simulink library "Steer_Rack_Wheel_Indep"  (R2025a)
settings: Solver=VariableStepAuto  StartTime=0.0  StopTime=10.0  RelTol=1e-3
undefined symbols (not defined in the file): Steer, Visual, X, Y, Z
libraries: sm_lib x10, nesl_utility x5, Driver_Systems x1, SteeringWheel x1, Vehicle_Inputs x1
Description:
  | Component of Simscape Vehicle Templates Library
  | 
  | Copyright 2018-2026 The MathWorks, Inc.
settings Model: Creator=smiller  LastModifiedBy=smiller
settings OptimizationCC: ReuseModelBlockBuffer=off
settings ModelReferenceCC: EnableRefExpFcnMdlSchedulingChecks=on
settings RTWCC: GPUComputeCapability=3.5

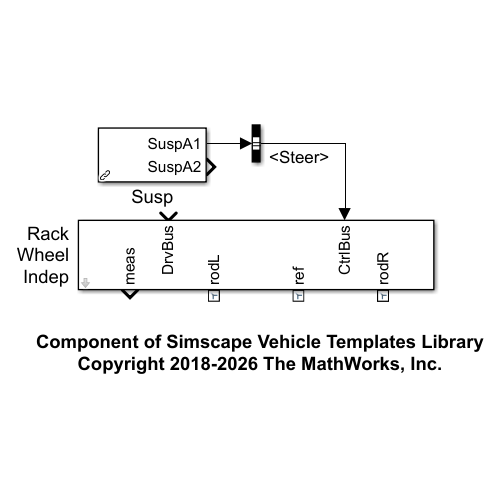
[thumbnail: Simulink's stored preview of the top-level diagram]
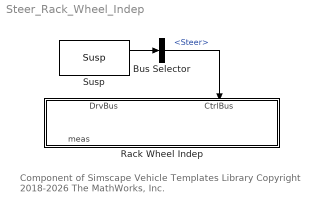
== system Steer_Rack_Wheel_Indep ==
  note: Component of Simscape Vehicle Templates Library
      | Copyright 2018-2026 The MathWorks, Inc.
  Bus Selector : BusSelector  OutputSignals=Steer
  Rack Wheel Indep : Subsystem  Tag=PublishSubsystem  VariantControl=Rack  mask(Steering System with Independent Steering Wheel and Rack Actuation){hp_wheel=Steer.Wheel.sMount.Value, wheel_axis_incl=Steer.Wheel.aAxis.Value, hp_mt_rack=Steer.Rack.sMount.Value, hp_out_rack=Steer.Rack.sOutboard.Value, Wheel=Steer.Wheel, rack_mass=Steer.Rack.m.Value, whl2rack_filter=1/Steer.Rack.fActuatorCutoff.Value, clr_rack=Visual.SteeringRack.clr, opc_rack=Visual.part.opc, radius_rack=Visual.SteeringRack.clr, clr_connhp=Visual.hp.clr, opc_connhp=Visual.hp.opc, size_connhp=Visual.hp.rad, clr_wheel=Visual.SteeringWheel.clr, opc_wheel=Visual.part.opc, DriverHuman=Steer.DriverHuman}
      mask prompts: hp_wheel "HP Wheel [xyz] (m)"; wheel_axis_incl "Wheel Axis Angle (rad)"; hp_mt_rack "HP Rack Mount [xyz] (m)"; hp_out_rack "HP Track Rod Inboard [xyz] (m)"; whl2rack_filter "Rack Motion Filter (sec)"; DriverHuman "Driver Human (structure)"
      mask help: Steering wheel angle and rack position are commanded independently by the control system. Specifying positions independently is suitable for steer-by-wire systems where the ratio of steering wheel angle to rack position ratio varies with vehicle conditions, such as vehicle speed. This model assumes the actuators are strong enough to achieve whatever positions are requested. Steering column shafts are not present.
      mask TypeOptions hp_wheel:
      | Ref to Wheel/Transform
      | HP Wheel/TranslationCartesianOffset
      mask TypeOptions hp_mt_rack:
      | Ref to Rack/Transform
      | HP Rack/TranslationCartesianOffset
      mask TypeOptions hp_out_rack: Rack/hp_out
      mask TypeOptions rack_mass: Rack/rack_mass
      mask TypeOptions whl2rack_filter: Physical Signal/InputFilterTimeConstant
      mask TypeOptions clr_rack: Rack/clr_rack
      mask TypeOptions opc_rack: Rack/opc_rack
      mask TypeOptions radius_rack: Rack/radius_rack
      mask TypeOptions clr_connhp:
      | Ref to Rack/Vis
      | Rack
      | Housing/GraphicDiffuseColor
      mask TypeOptions opc_connhp:
      | Ref to Rack/Vis
      | Rack
      | Housing/GraphicOpacity
      mask TypeOptions size_connhp:
      | Ref to Rack/Vis
      | Rack
      | Housing/SphereRadius
      mask TypeOptions clr_wheel: Wheel/clr_wheel
      mask TypeOptions opc_wheel: Wheel/opc_wheel
      mask DialogControl cont_steer Prompt: Steer
      mask DialogControl grp_strparts Prompt: Parts
      mask DialogControl text_strparts_len Prompt: Length/Radius (m)
      mask DialogControl text_strparts_mass Prompt: Mass (kg)
      mask DialogControl text_strparts_wheel Prompt: Wheel
      mask DialogControl text_strparts_wheel_m Prompt: <CAD file>
      mask DialogControl text_strparts_rack Prompt: Rack
      mask DialogControl text_strparts_rack_len Prompt: <HP Rod Inboard>
      mask DialogControl grp_whl2rack Prompt: Wheel to Rack
      mask DialogControl cont_vis_steer Prompt: Visualization
      mask DialogControl text_steer_vis_clr Prompt: Color [RGB]
      mask DialogControl text_steer_vis_opc Prompt: Opac. (0-1)
      mask DialogControl text_steer_vis_size Prompt: Size (m)
      mask DialogControl text_steer_vis_rack Prompt: Rack
      mask DialogControl text_steer_vis_connhp Prompt: Connections, HP
      mask DialogControl text_steer_vis_wheel Prompt: Wheel
      mask DialogControl text_wheel_size Prompt: <CAD File>
      mask DialogControl cont_driver_human Prompt: Driver Human
  Susp : Vehicle_Inputs/Control Bus/Susp  SystemSampleTime=-1  VariantActivationTime=update diagram  EmptyChoice=off  PassThrough=off  PassThroughVariantControl=(default)  EmptyChoiceVariantControl=(default)  AllowFlexibleInterface=on  Latency=0  AutoFrameSizeCalculation=off
  wires:
  Bus Selector/1 -> Rack Wheel Indep/2(CtrlBus)  "<Steer>"
  Susp/1 -> Bus Selector/1

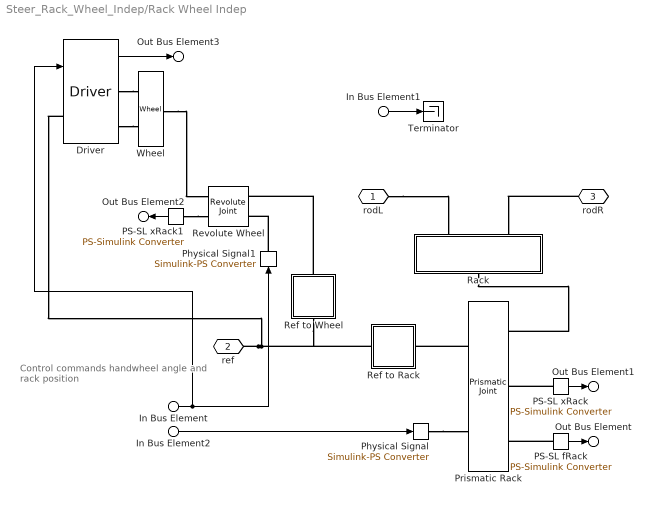
== system Steer_Rack_Wheel_Indep/Rack Wheel Indep ==
  note: Control commands handwheel
      | angle and rack position
  In Bus Element1 : Inport  PortName=DrvBus  Element=aSteerWheel
  In Bus Element : Inport  Port=2  PortName=CtrlBus  Element=aSteerWheel
  In Bus Element2 : Inport  Port=2  PortName=CtrlBus  Element=xRack
  Driver : Driver_Systems/Driver  LabelModeActiveChoice=Human  DriverHuman=DriverHuman  VariantLabel=DriverHuman.class.Value
      settings: AttributesFormatString=%<LabelModeActiveChoice>
  PS-SL fRack : nesl_utility/PS-Simulink Converter  PhysicalDomain=network_engine_domain  SubClassName=ps_output  LeftPortType=input  RightPortType=output  PseudoPeriodic=off  Frequencies=[]  VectorFormat=1-D array  Unit=1  AffineConversion=off
  PS-SL xRack : nesl_utility/PS-Simulink Converter  PhysicalDomain=network_engine_domain  SubClassName=ps_output  LeftPortType=input  RightPortType=output  PseudoPeriodic=off  Frequencies=[]  VectorFormat=1-D array  Unit=1  AffineConversion=off
  PS-SL xRack1 : nesl_utility/PS-Simulink Converter  PhysicalDomain=network_engine_domain  SubClassName=ps_output  LeftPortType=input  RightPortType=output  PseudoPeriodic=off  Frequencies=[]  VectorFormat=1-D array  Unit=rad  AffineConversion=off
  Physical Signal : nesl_utility/Simulink-PS Converter  PhysicalDomain=network_engine_domain  SubClassName=ps_input  LeftPortType=input  RightPortType=output  PseudoPeriodic=off  Frequencies=[]  NoiseDistribution=none  NoiseParameters=[]  Unit=m  AffineConversion=off  FilteringAndDerivatives=filter  SimscapeFilterOrder=2  InputFilterTimeConstant=whl2rack_filter  UdotUserProvided=0
      settings: AttributesFormatString=|
      | Filter Time Constant
      | %<InputFilterTimeConstant> sec
  Physical Signal1 : nesl_utility/Simulink-PS Converter  PhysicalDomain=network_engine_domain  SubClassName=ps_input  LeftPortType=input  RightPortType=output  PseudoPeriodic=off  Frequencies=[]  NoiseDistribution=none  NoiseParameters=[]  Unit=rad  AffineConversion=off  FilteringAndDerivatives=filter  SimscapeFilterOrder=2  InputFilterTimeConstant=whl2rack_filter  UdotUserProvided=0
      settings: AttributesFormatString=|
      | Filter Time Constant
      | %<InputFilterTimeConstant> sec
  Prismatic Rack : sm_lib/Joints/Prismatic Joint  JointMode=Normal  CompositeWrenchDir=FollowerOnBase  CompositeWrenchFrame=BaseFrame  SenseConstraintForce=off  SenseConstraintTorque=off  SenseTotalForce=off  SenseTotalTorque=off  PositionTargetSpecify=on  PositionTargetPriority=Low  PositionTargetValue=0  PositionTargetValueUnits=m  VelocityTargetSpecify=off  VelocityTargetPriority=High  VelocityTargetValue=0  VelocityTargetValueUnits=m/s  EquilibriumPosition=0  EquilibriumPositionUnits=m  SpringStiffness=0  SpringStiffnessUnits=N/m  DampingCoefficient=1e5*0  DampingCoefficientUnits=N/(m/s)  LowerLimitSpecify=off  LowerLimitBound=-1  LowerLimitBoundUnits=m  LowerLimitStiffness=1e6  LowerLimitStiffnessUnits=N/m  LowerLimitDamping=1e3  LowerLimitDampingUnits=N/(m/s)  LowerLimitTransitionRegionWidth=1e-4  LowerLimitTransitionRegionWidthUnits=m  UpperLimitSpecify=off  UpperLimitBound=1  UpperLimitBoundUnits=m  UpperLimitStiffness=1e6  UpperLimitStiffnessUnits=N/m  UpperLimitDamping=1e3  UpperLimitDampingUnits=N/(m/s)  UpperLimitTransitionRegionWidth=1e-4  UpperLimitTransitionRegionWidthUnits=m  TorqueActuationMode=ComputedTorque  MotionActuationMode=InputMotion  SensePosition=on  SenseVelocity=off  SenseAcceleration=off  SenseTorqueForce=on  SenseLowerLimitTorqueForce=off  SenseUpperLimitTorqueForce=off
  Rack : Subsystem  mask{hp_out=hp_out_rack, rack_mass=rack_mass, clr_rack=clr_rack, opc_rack=opc_rack, radius_rack=radius_rack}
      mask prompts: hp_out "HP Track Rod Inboard [xyz] (m)"; rack_mass "Mass (kg)"
      mask init:
      | rack_length = norm(hp_out-hp_out.*[1 -1 1]);
      mask TypeOptions rack_mass: Rack/Mass
      mask TypeOptions clr_rack: Rack/GraphicDiffuseColor
      mask TypeOptions opc_rack: Rack/GraphicOpacity
      mask TypeOptions radius_rack: Rack/CylinderRadius
      mask DialogControl cont_rack Prompt: Rack
      mask DialogControl text_rack_clr Prompt: Color [RGB]
      mask DialogControl text_rack_opc Prompt: Opac. (0-1)
      mask DialogControl text_rack_size Prompt: Size (m)
      mask DialogControl text_rack_rack Prompt: Rack
  Ref to Rack : Subsystem
  Ref to Wheel : Subsystem
  Revolute Wheel : sm_lib/Joints/Revolute Joint  JointMode=Normal  CompositeWrenchDir=FollowerOnBase  CompositeWrenchFrame=BaseFrame  SenseConstraintForce=off  SenseConstraintTorque=off  SenseTotalForce=off  SenseTotalTorque=off  PositionTargetSpecify=on  PositionTargetPriority=Low  PositionTargetValue=0  PositionTargetValueUnits=deg  VelocityTargetSpecify=off  VelocityTargetPriority=High  VelocityTargetValue=0  VelocityTargetValueUnits=deg/s  EquilibriumPosition=0  EquilibriumPositionUnits=deg  SpringStiffness=0  SpringStiffnessUnits=N*m/deg  DampingCoefficient=0  DampingCoefficientUnits=N*m/(deg/s)  LowerLimitSpecify=off  LowerLimitBound=-90  LowerLimitBoundUnits=deg  LowerLimitStiffness=1e4  LowerLimitStiffnessUnits=N*m/deg  LowerLimitDamping=10  LowerLimitDampingUnits=N*m/(deg/s)  LowerLimitTransitionRegionWidth=0.1  LowerLimitTransitionRegionWidthUnits=deg  UpperLimitSpecify=off  UpperLimitBound=90  UpperLimitBoundUnits=deg  UpperLimitStiffness=1e4  UpperLimitStiffnessUnits=N*m/deg  UpperLimitDamping=10  UpperLimitDampingUnits=N*m/(deg/s)  UpperLimitTransitionRegionWidth=0.1  UpperLimitTransitionRegionWidthUnits=deg  TorqueActuationMode=ComputedTorque  MotionActuationMode=InputMotion  SensePosition=on  SenseVelocity=off  SenseAcceleration=off  SenseTorqueForce=off  SenseLowerLimitTorqueForce=off  SenseUpperLimitTorqueForce=off
  Terminator : Terminator
  Wheel : SteeringWheel/Wheel  LabelModeActiveChoice=Sedan  VariantLabel=Wheel.class.Value
  rodL : PMIOPort  Side=Right
  ref : PMIOPort  Port=2  Side=Right
  rodR : PMIOPort  Port=3  Side=Right
  Out Bus Element : Outport  VectorParamsAs1DForOutWhenUnconnected=off  PortName=meas  Element=FRack
  Out Bus Element1 : Outport  VectorParamsAs1DForOutWhenUnconnected=off  PortName=meas  Element=xRack
  Out Bus Element2 : Outport  VectorParamsAs1DForOutWhenUnconnected=off  PortName=meas  Element=aWheel
  Out Bus Element3 : Outport  VectorParamsAs1DForOutWhenUnconnected=off  PortName=meas  Element=Driver
  wires:
  In Bus Element1/1 -> Terminator/1
  Driver/1 -> Out Bus Element3/1
  PS-SL xRack1/1 -> Out Bus Element2/1
  In Bus Element/1 -> Driver/1, Physical Signal1/1
  In Bus Element2/1 -> Physical Signal/1
  PS-SL fRack/1 -> Out Bus Element/1
  PS-SL xRack/1 -> Out Bus Element1/1
  connections:
  Driver/RConn2 -- Wheel/RConn2
  Driver/RConn1 -- Wheel/RConn1
  PS-SL xRack1/LConn1 -- Revolute Wheel/RConn2
  rodR/RConn1 -- Rack/LConn2
  rodL/RConn1 -- Rack/LConn1
  Prismatic Rack/LConn1 -- Ref to Rack/RConn1
  Ref to Wheel/RConn1 -- Revolute Wheel/LConn1
  Physical Signal1/RConn1 -- Revolute Wheel/LConn2
  Wheel/LConn1 -- Revolute Wheel/RConn1
  PS-SL xRack/LConn1 -- Prismatic Rack/RConn2
  Physical Signal/RConn1 -- Prismatic Rack/LConn2
  Rack/RConn1 -- Prismatic Rack/RConn1
  ref/RConn1 -- Driver/LConn1 -- Ref to Rack/LConn1 -- Ref to Wheel/LConn1
  PS-SL fRack/LConn1 -- Prismatic Rack/RConn3

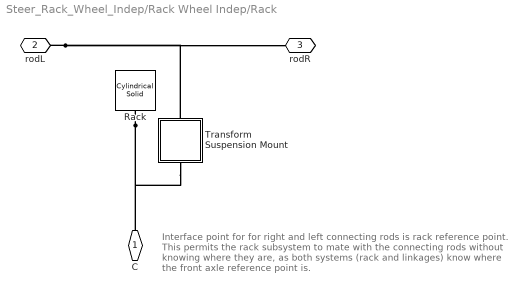
== system Steer_Rack_Wheel_Indep/Rack Wheel Indep/Rack ==
  note: Interface point for for right and left connecting rods is rack reference point. This permits the rack subsystem to mate with the connecting rods without knowing where they are, as both systems (rack and linkages) know where the front axle reference point is.
  Rack : sm_lib/Body Elements/Cylindrical Solid  CylinderRadius=radius_rack  CylinderRadiusUnits=m  CylinderLength=rack_length  CylinderLengthUnits=m  ExportEntireGeometry=off  InertiaType=CalculateFromGeometry  BasedOnType=Mass  Density=7000  DensityUnits=kg/m^3  Mass=rack_mass  MassUnits=kg  CenterOfMass=[0 0 0]  CenterOfMassUnits=m  MomentsOfInertia=[1 1 1]  MomentsOfInertiaUnits=kg*m^2  ProductsOfInertia=[0 0 0]  ProductsOfInertiaUnits=kg*m^2  GraphicType=FromGeometry  MarkerShape=Sphere  MarkerSize=10  GraphicVisPropType=SimpleVisualProperties  GraphicDiffuseColor=clr_rack  GraphicOpacity=opc_rack  GraphicSpecularColor=[0.5 0.5 0.5 1.0]  GraphicAmbientColor=[0.15 0.15 0.15 1.0]  GraphicEmissiveColor=[0.0 0.0 0.0 1.0]  GraphicShininess=75  DoExposeReferenceFrame=on  SerializedFrames=<Frames/>
  Transform Suspension Mount : Subsystem
  C : PMIOPort  Side=Right
  rodL : PMIOPort  Port=2  Side=Left
  rodR : PMIOPort  Port=3  Side=Left
  connections:
  rodL/RConn1 -- rodR/RConn1 -- Transform Suspension Mount/LConn1
  Rack/RConn1 -- Transform Suspension Mount/RConn1 -- C/RConn1

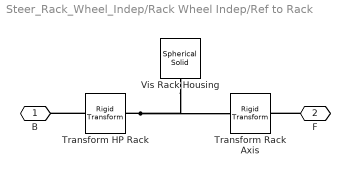
== system Steer_Rack_Wheel_Indep/Rack Wheel Indep/Ref to Rack ==
  Transform HP Rack : sm_lib/Frames and Transforms/Rigid Transform  RotationMethod=None  FollAlignAxisA=+X  BaseAlignAxisA=+Y  FollAlignAxisB=+Y  BaseAlignAxisB=+Z  RotationStandardAxis=+Z  RotationAngle=0.0  RotationAngleUnits=deg  RotationArbitraryAxis=[0 0 1]  RotationSequenceAxes=FollowerAxes  RotationSequence=XYX  RotationSequenceAngles=[0 0 0]  RotationSequenceAnglesUnits=deg  RotationMatrix=[1 0 0; 0 1 0; 0 0 1]  Quaternion=[1 0 0 0]  TranslationMethod=Cartesian  TranslationCartesianOffset=hp_mt_rack  TranslationCartesianOffsetUnits=m  TranslationStandardAxis=+Z  TranslationStandardOffset=0  TranslationStandardOffsetUnits=m  TranslationROffset=0  TranslationROffsetUnits=m  TranslationThetaOffset=0  TranslationThetaOffsetUnits=deg  TranslationZOffset=0  TranslationZOffsetUnits=m
  Transform Rack Axis : sm_lib/Frames and Transforms/Rigid Transform  RotationMethod=AlignedAxes  FollAlignAxisA=+Y  BaseAlignAxisA=-Z  FollAlignAxisB=+X  BaseAlignAxisB=+X  RotationStandardAxis=+Z  RotationAngle=0  RotationAngleUnits=deg  RotationArbitraryAxis=[0 0 1]  RotationSequenceAxes=FollowerAxes  RotationSequence=XYX  RotationSequenceAngles=[0 0 0]  RotationSequenceAnglesUnits=deg  RotationMatrix=[0 0 -1;0 1 0;1 0 0]  Quaternion=[1 0 0 0]  TranslationMethod=None  TranslationCartesianOffset=[0 0 0]  TranslationCartesianOffsetUnits=m  TranslationStandardAxis=+Z  TranslationStandardOffset=0  TranslationStandardOffsetUnits=m  TranslationROffset=0  TranslationROffsetUnits=m  TranslationThetaOffset=0  TranslationThetaOffsetUnits=deg  TranslationZOffset=0  TranslationZOffsetUnits=m
  Vis Rack Housing : sm_lib/Body Elements/Spherical Solid  SphereRadius=size_connhp  SphereRadiusUnits=m  ExportEntireGeometry=off  InertiaType=CalculateFromGeometry  BasedOnType=Density  Density=1000  DensityUnits=kg/m^3  Mass=1  MassUnits=kg  CenterOfMass=[0 0 0]  CenterOfMassUnits=m  MomentsOfInertia=[1 1 1]  MomentsOfInertiaUnits=kg*m^2  ProductsOfInertia=[0 0 0]  ProductsOfInertiaUnits=kg*m^2  GraphicType=FromGeometry  MarkerShape=Sphere  MarkerSize=10  GraphicVisPropType=SimpleVisualProperties  GraphicDiffuseColor=clr_connhp  GraphicOpacity=opc_connhp  GraphicSpecularColor=[0.5 0.5 0.5 1.0]  GraphicAmbientColor=[0.15 0.15 0.15 1.0]  GraphicEmissiveColor=[0.0 0.0 0.0 1.0]  GraphicShininess=75  DoExposeReferenceFrame=on  SerializedFrames=<Frames/>
  B : PMIOPort  Side=Left
  F : PMIOPort  Port=2  Side=Right
  connections:
  F/RConn1 -- Transform Rack Axis/RConn1
  Transform HP Rack/LConn1 -- B/RConn1
  Transform HP Rack/RConn1 -- Transform Rack Axis/LConn1 -- Vis Rack Housing/RConn1

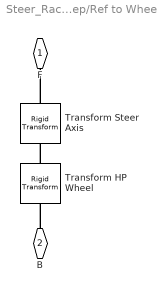
== system Steer_Rack_Wheel_Indep/Rack Wheel Indep/Ref to Wheel ==
  Transform HP Wheel : sm_lib/Frames and Transforms/Rigid Transform  RotationMethod=None  FollAlignAxisA=+X  BaseAlignAxisA=+Y  FollAlignAxisB=+Y  BaseAlignAxisB=+Z  RotationStandardAxis=+Z  RotationAngle=0.0  RotationAngleUnits=deg  RotationArbitraryAxis=[0 0 1]  RotationSequenceAxes=FollowerAxes  RotationSequence=XYX  RotationSequenceAngles=[0 0 0]  RotationSequenceAnglesUnits=deg  RotationMatrix=[1 0 0; 0 1 0; 0 0 1]  Quaternion=[1 0 0 0]  TranslationMethod=Cartesian  TranslationCartesianOffset=hp_wheel  TranslationCartesianOffsetUnits=m  TranslationStandardAxis=+Z  TranslationStandardOffset=0  TranslationStandardOffsetUnits=m  TranslationROffset=0  TranslationROffsetUnits=m  TranslationThetaOffset=0  TranslationThetaOffsetUnits=deg  TranslationZOffset=0  TranslationZOffsetUnits=m
  Transform Steer Axis : sm_lib/Frames and Transforms/Rigid Transform  RotationMethod=StandardAxis  FollAlignAxisA=+X  BaseAlignAxisA=+Y  FollAlignAxisB=+Y  BaseAlignAxisB=+Z  RotationStandardAxis=+Y  RotationAngle=-pi/2+wheel_axis_incl  RotationAngleUnits=rad  RotationArbitraryAxis=[0 0 1]  RotationSequenceAxes=FollowerAxes  RotationSequence=XYX  RotationSequenceAngles=[0 0 0]  RotationSequenceAnglesUnits=deg  RotationMatrix=[1 0 0; 0 1 0; 0 0 1]  Quaternion=[1 0 0 0]  TranslationMethod=None  TranslationCartesianOffset=[0 0 0]  TranslationCartesianOffsetUnits=m  TranslationStandardAxis=+Z  TranslationStandardOffset=0  TranslationStandardOffsetUnits=m  TranslationROffset=0  TranslationROffsetUnits=m  TranslationThetaOffset=0  TranslationThetaOffsetUnits=deg  TranslationZOffset=0  TranslationZOffsetUnits=m
  F : PMIOPort  Side=Right
  B : PMIOPort  Port=2  Side=Left
  connections:
  Transform Steer Axis/RConn1 -- F/RConn1
  B/RConn1 -- Transform HP Wheel/LConn1
  Transform HP Wheel/RConn1 -- Transform Steer Axis/LConn1

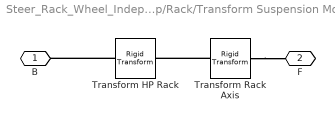
== system Steer_Rack_Wheel_Indep/Rack Wheel Indep/Rack/Transform Suspension Mount ==
  Transform HP Rack : sm_lib/Frames and Transforms/Rigid Transform  RotationMethod=None  FollAlignAxisA=+X  BaseAlignAxisA=+Y  FollAlignAxisB=+Y  BaseAlignAxisB=+Z  RotationStandardAxis=+Z  RotationAngle=0.0  RotationAngleUnits=deg  RotationArbitraryAxis=[0 0 1]  RotationSequenceAxes=FollowerAxes  RotationSequence=XYX  RotationSequenceAngles=[0 0 0]  RotationSequenceAnglesUnits=deg  RotationMatrix=[1 0 0; 0 1 0; 0 0 1]  Quaternion=[1 0 0 0]  TranslationMethod=Cartesian  TranslationCartesianOffset=hp_mt_rack  TranslationCartesianOffsetUnits=m  TranslationStandardAxis=+Z  TranslationStandardOffset=0  TranslationStandardOffsetUnits=m  TranslationROffset=0  TranslationROffsetUnits=m  TranslationThetaOffset=0  TranslationThetaOffsetUnits=deg  TranslationZOffset=0  TranslationZOffsetUnits=m
  Transform Rack Axis : sm_lib/Frames and Transforms/Rigid Transform  RotationMethod=AlignedAxes  FollAlignAxisA=+Y  BaseAlignAxisA=-Z  FollAlignAxisB=+X  BaseAlignAxisB=+X  RotationStandardAxis=+Z  RotationAngle=0  RotationAngleUnits=deg  RotationArbitraryAxis=[0 0 1]  RotationSequenceAxes=FollowerAxes  RotationSequence=XYX  RotationSequenceAngles=[0 0 0]  RotationSequenceAnglesUnits=deg  RotationMatrix=[0 0 -1;0 1 0;1 0 0]  Quaternion=[1 0 0 0]  TranslationMethod=None  TranslationCartesianOffset=[0 0 0]  TranslationCartesianOffsetUnits=m  TranslationStandardAxis=+Z  TranslationStandardOffset=0  TranslationStandardOffsetUnits=m  TranslationROffset=0  TranslationROffsetUnits=m  TranslationThetaOffset=0  TranslationThetaOffsetUnits=deg  TranslationZOffset=0  TranslationZOffsetUnits=m
  B : PMIOPort  Side=Left
  F : PMIOPort  Port=2  Side=Right
  connections:
  Transform Rack Axis/RConn1 -- F/RConn1
  Transform HP Rack/LConn1 -- B/RConn1
  Transform Rack Axis/LConn1 -- Transform HP Rack/RConn1
